simulink model "DPS_LC"  (R2025b)
settings: Solver=FixedStepAuto  StartTime=0.0  StopTime=1  FixedStep=1e-7  RelTol=1e-3
undefined symbols (not defined in the file): Ion, Lithium
libraries: spsVoltageMeasurementLib x5, spsCurrentMeasurementLib x4, spsIGBTDiodeLib x4, spsMosfetLib x4, spsSeriesRLCBranchLib x4, spsDCVoltageSourceLib x2, spsMeanLib x2, spsBatteryLib x1, spsLinearTransformerLib x1, sps_lib x1
settings Model: Creator=photortist  LastModifiedBy=Admin

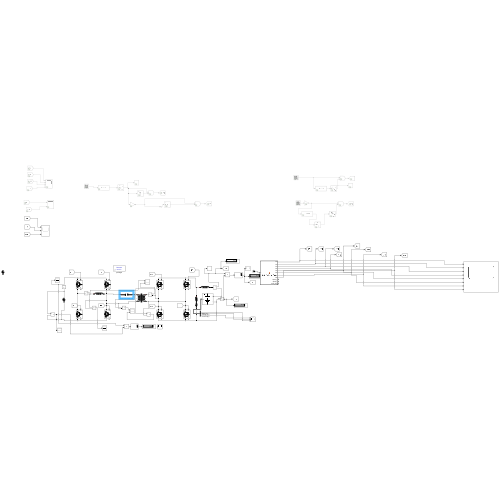
[thumbnail: Simulink's stored preview of the top-level diagram]
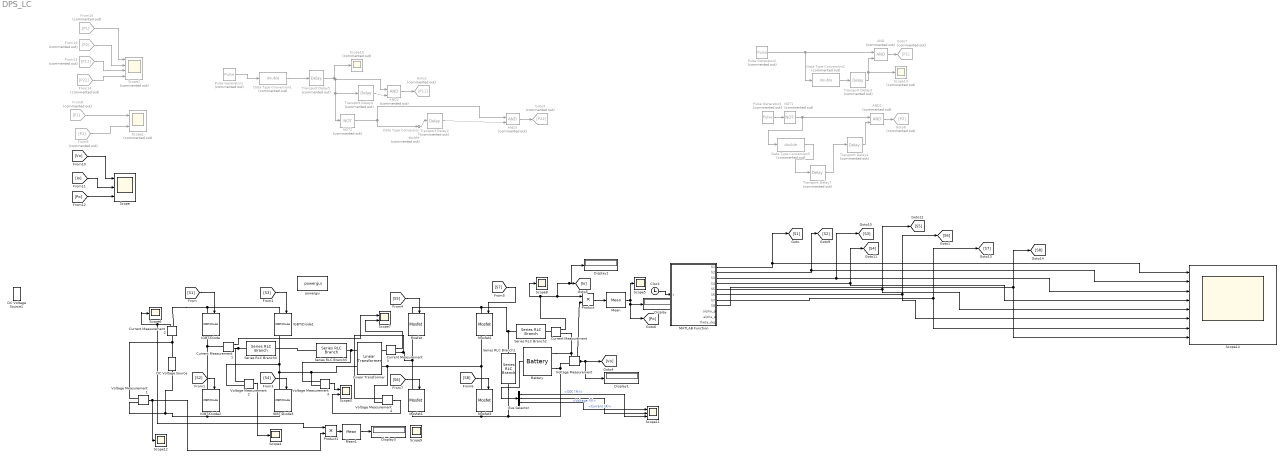
== system DPS_LC ==
  AND{,1..3} (4 alike) : Logic  Commented=on  IconShape=distinctive  AllPortsSameDT=off  OutDataTypeStr=boolean
  Battery : spsBatteryLib/Battery  BatType=Lithium-Ion  NomV=24  NomQ=100  SOC=10  Batt_Tr=0.1  PresetModel=on  MaxQ=100  MinV=18  FullV=27.9357  Dis_rate=43.4783  R=0.0024  Normal_OP=90.4348  expZone="[25.9293      4.91304]"
  Bus Selector : BusSelector  OutputSignals=SOC (%),Voltage (V),Current (A)
  Clock : Clock
  Current Measurement{,1..3} (4 alike) : spsCurrentMeasurementLib/Current Measurement  PhasorSimulation=off  OutputType=Complex  PSBequivalent=0
  DC Voltage Source : spsDCVoltageSourceLib/DC Voltage Source  Amplitude=504  Measurements=None
  DC Voltage Source1 : spsDCVoltageSourceLib/DC Voltage Source  Amplitude=504  Measurements=None
  Data Type Conversion{1..3,5} (4 alike) : DataTypeConversion  Commented=on  OutDataTypeStr=double  SaturateOnIntegerOverflow=off  RndMeth=Floor
  Display{,1..3} (4 alike) : Display
  From13 : From  Commented=on  GotoTag=P11
  From14 : From  Commented=on  GotoTag=P22
  From15 : From  Commented=on  GotoTag=P1
  From16 : From  Commented=on  GotoTag=P2
  From8 : From  Commented=on  GotoTag=P1
  From9 : From  Commented=on  GotoTag=P2
  Goto2 : Goto  Commented=on  GotoTag=P11
  Goto3 : Goto  Commented=on  GotoTag=P22
  Goto7 : Goto  Commented=on  GotoTag=P1
  Goto8 : Goto  Commented=on  GotoTag=P2
  IGBT/Diode{,1..3} (4 alike) : spsIGBTDiodeLib/IGBT//Diode  Ron=1e-4  Rs=1e5  Cs=inf  Measurements=on
  Linear Transformer : spsLinearTransformerLib/Linear Transformer  UNITS=SI  NominalPower=[ 3000 30000 ]  winding1=[504 0 0]  winding2=[28 0 0]  ThreeWindings=off  winding3=[3.15e+05 0.7938 0.084225]  RmLm="[5000  0.05]"  Measurements=None  DataType=on
  MATLAB Function : MATLAB Function  TreatAsAtomicUnit=on
  Mean : spsMeanLib/Mean  Freq=30e3  Vinit=0  Ts=0
  Mean1 : spsMeanLib/Mean  Freq=30e3  Vinit=0  Ts=0
  Mosfet{,1..3} (4 alike) : spsMosfetLib/Mosfet  Ron=1e-4  Lon=0  Rd=0.01  Vfd=0  IC=0  Rs=1e5  Cs=inf  Measurements=on
  NOT1 : Logic  Commented=on  Operator=NOT  IconShape=distinctive  AllPortsSameDT=off  OutDataTypeStr=boolean
  NOT2 : Logic  Commented=on  Operator=NOT  IconShape=distinctive  AllPortsSameDT=off  OutDataTypeStr=boolean
  Product : Product
  Product1 : Product
  Pulse Generator1 : DiscretePulseGenerator  Commented=on  PulseType=Time based  Period=1/30000  PulseWidth=50  PhaseDelay=16.67e-6
  Pulse Generator2 : DiscretePulseGenerator  Commented=on  PulseType=Time based  Period=1/30000  PulseWidth=50  VectorParams1D=off
  Pulse Generator4 : DiscretePulseGenerator  Commented=on  PulseType=Time based  Period=1/30000  PulseWidth=50  VectorParams1D=off
  Scope : Scope  NumInputPorts=3
      settings: Title=Output Voltage  ActiveDisplayYMinimum=-3.1740035321909232  ActiveDisplayYMaximum=28.566031789718316
  Scope1 : Scope  Commented=on  NumInputPorts=2
      settings: ActiveDisplayYMinimum=-1  ActiveDisplayYMaximum=1
  Scope10 : Scope  Commented=on
      settings: ActiveDisplayYMinimum=-0.12499999999999997  ActiveDisplayYMaximum=1.125  DataLoggingVariableName=ScopeData10
  Scope11 : Scope  NumInputPorts=3
      settings: ActiveDisplayYMinimum=-34.642469319088491  ActiveDisplayYMaximum=273.73320486745138  DataLoggingVariableName=ScopeData11
  Scope{4..6,8..9,12} (6 alike) : Scope
      Scope12 settings: ActiveDisplayYMinimum=404  ActiveDisplayYMaximum=604  DataLoggingVariableName=ScopeData12
      Scope4 settings: ActiveDisplayYMinimum=-630.02715891615526  ActiveDisplayYMaximum=630.02739265310572  DataLoggingVariableName=ScopeData4
      Scope5 settings: ActiveDisplayYMinimum=-393.10954952872225  ActiveDisplayYMaximum=3537.9859457585012  DataLoggingVariableName=ScopeData5
      Scope6 settings: ActiveDisplayYMinimum=-23.635845868791428  ActiveDisplayYMaximum=24.862575673067333  DataLoggingVariableName=ScopeData6
      Scope8 settings: ActiveDisplayYMinimum=-843.85888992789546  ActiveDisplayYMaximum=389.64380681826373  DataLoggingVariableName=ScopeData8
      Scope9 settings: ActiveDisplayYMinimum=-44.04044538673373  ActiveDisplayYMaximum=46.396500117844894  DataLoggingVariableName=ScopeData9
  Scope13 : Scope  Commented=on
      settings: ActiveDisplayYMinimum=-0.12499999999999997  ActiveDisplayYMaximum=1.125  DataLoggingVariableName=ScopeData13
  Scope14 : Scope  NumInputPorts=8
      settings: ActiveDisplayYMinimum=-0.12499999999999997  ActiveDisplayYMaximum=1.125  DataLoggingVariableName=ScopeData14
  Scope2 : Scope  Commented=on  NumInputPorts=4
      settings: ActiveDisplayYMinimum=-0.12499999999999997  ActiveDisplayYMaximum=1.125  DataLoggingVariableName=ScopeData2
  Scope3 : Scope  NumInputPorts=2
      settings: ActiveDisplayYMinimum=-1348.3166244930978  ActiveDisplayYMaximum=1342.78051192566  DataLoggingVariableName=ScopeData3
  Scope7 : Scope  NumInputPorts=2
      settings: ActiveDisplayYMinimum=-55.436527647349514  ActiveDisplayYMaximum=40.992607448281404  DataLoggingVariableName=ScopeData7
  Series RLC Branch1 : spsSeriesRLCBranchLib/Series RLC Branch  LConnTagsString=__new0  RConnTagsString=__new0  BranchType=RC  Resistance=0.2  Inductance=1e-3  SetiL0=off  InitialCurrent=0  Capacitance=0.226e-6  Setx0=off  InitialVoltage=0  Measurements=None
  Series RLC Branch2 : spsSeriesRLCBranchLib/Series RLC Branch  LConnTagsString=__new0  RConnTagsString=__new0  BranchType=L  Resistance=7  Inductance=0.5e-6  SetiL0=off  InitialCurrent=0  Capacitance=1e-6  Setx0=off  InitialVoltage=0  Measurements=None
  Series RLC Branch4 : spsSeriesRLCBranchLib/Series RLC Branch  LConnTagsString=__new0  RConnTagsString=__new0  BranchType=L  Resistance=1  Inductance=40e-6  SetiL0=off  InitialCurrent=0  Capacitance=1e-6  Setx0=off  InitialVoltage=0  Measurements=None
  Series RLC Branch5 : spsSeriesRLCBranchLib/Series RLC Branch  LConnTagsString=__new0  RConnTagsString=__new0  BranchType=C  Resistance=0.01  Inductance=350e-6  SetiL0=off  InitialCurrent=0  Capacitance=80.8e-6  Setx0=off  InitialVoltage=0  Measurements=None
  Transport Delay{2..4,6..7} (5 alike) : TransportDelay  Commented=on  DelayTime=0.2e-6
  Transport Delay5 : TransportDelay  Commented=on  DelayTime=16.67e-6
  Voltage Measurement{,1..4} (5 alike) : spsVoltageMeasurementLib/Voltage Measurement  PhasorSimulation=off  OutputType=Complex  PSBequivalent=0
  powergui : sps_lib/powergui  Priority=1  SimulationMode=Discrete  SampleTime=0.1e-6  frequency=60  Iterations=50  frequencyindice=0  Pbase=100e6  ErrMax=1e-4  UnitsV=kV  UnitsW=MW  buscounter=0  FunctionMessages=off  echomessages=off  EnableUseOfTLC=off  CurrentSourceSwitches=off  DisableSnubberDevices=off  DisableRonSwitches=off  DisableVfSwitches=off  DisplayEquations=off  AutomaticDiscreteSolvers=off  SolverType=Tustin/Backward Euler (TBE)  Interpol=off  ExternalGateDelay=off  methode=off  Ts=100  x0status=blocks  SPID=on  SwTol=0  HookPort=off  NonlinearTolerance=1e-4  nMaxIteration=100  ContinueOnMaxIteration=off  RestoreLinks=warning  ResistiveCurrentMeasurement=off  Frange=[0:2:500]  Ylog=off  Xlog=on  ShowGrid=off  save=off  variable=ZData  structure=0  ZoomFFT=off  StartTime=0.0  cycles=1  DisplayStyle=1  fundamental=60  FreqAxis=off  MaxFrequency=1000  frequencyindicesteady=1  RmsSteady=1  display=off
  wires:
  Current Measurement2/1 -> Product1/1, Scope6/1
  Product/1 -> Mean/1
  [Vo] -> Scope/1
  [S2] -> IGBT/Diode2/1
  [S4] -> IGBT/Diode3/1
  [S6] -> Mosfet1/1
  Mean1/1 -> Display3/1
  Voltage Measurement1/1 -> Scope12/1, Product1/2
  From8/1 -> Scope1/1
  [S3] -> IGBT/Diode1/1
  From9/1 -> Scope1/2
  Current Measurement3/1 -> Scope7/2
  Voltage Measurement2/1 -> Scope4/1
  From14/1 -> Scope2/4
  [S8] -> Mosfet3/1
  Pulse Generator1/1 -> Data Type Conversion1/1
  Current Measurement/1 -> Scope8/1, Product/1, Display2/1, [Io]
  From16/1 -> Scope2/2
  [Io] -> Scope/2
  Mean/1 -> [Po], Display/1, Scope5/1
  [S7] -> Mosfet2/1
  Voltage Measurement3/1 -> Scope3/1
  [S1] -> IGBT/Diode/1
  From15/1 -> Scope2/1
  From13/1 -> Scope2/3
  Product1/1 -> Mean1/1
  Current Measurement1/1 -> Scope7/1
  [S5] -> Mosfet/1
  Voltage Measurement/1 -> Product/2, [Vo], Display1/1
  [Po] -> Scope/3
  Data Type Conversion2/1 -> Transport Delay3/1
  Pulse Generator2/1 -> Data Type Conversion2/1, AND/1
  Transport Delay3/1 -> Scope13/1, AND/2
  Transport Delay4/1 -> AND1/2
  Pulse Generator4/1 -> NOT1/1
  NOT1/1 -> Data Type Conversion3/1, AND1/1
  AND/1 -> Goto7/1
  AND1/1 -> Goto8/1
  NOT2/1 -> AND3/1, Data Type Conversion5/1
  Data Type Conversion1/1 -> Transport Delay5/1
  AND2/1 -> Goto2/1
  Transport Delay6/1 -> AND2/2
  Data Type Conversion5/1 -> Transport Delay2/1
  Transport Delay2/1 -> AND3/2
  AND3/1 -> Goto3/1
  Transport Delay5/1 -> AND2/1, NOT2/1, Transport Delay6/1, Scope10/1
  Data Type Conversion3/1 -> Transport Delay7/1
  Transport Delay7/1 -> Transport Delay4/1
  Voltage Measurement4/1 -> Scope3/2
  Battery/1 -> Bus Selector/1
  Bus Selector/1 -> Scope11/3  "<SOC (%)>"
  Bus Selector/2 -> Scope11/2  "<Voltage (V)>"
  Bus Selector/3 -> Scope11/1  "<Current (A)>"
  MATLAB Function/7(S7) -> [S7], Scope14/7
  MATLAB Function/6(S6) -> [S6], Scope14/6
  MATLAB Function/8(S8) -> Scope14/8, [S8]
  MATLAB Function/3(S3) -> [S3], Scope14/3
  MATLAB Function/5(S5) -> Scope14/5, [S5]
  MATLAB Function/1(S1) -> [S1], Scope14/1
  MATLAB Function/2(S2) -> [S2], Scope14/2
  MATLAB Function/4(S4) -> Scope14/4, [S4]
  Clock/1 -> MATLAB Function/1(t)
  connections:
  Current Measurement2/LConn1 -- DC Voltage Source/RConn1 -- Voltage Measurement1/LConn1
  Current Measurement3/RConn1 -- Mosfet1/LConn1 -- Mosfet/RConn1 -- Voltage Measurement4/LConn1
  Current Measurement1/RConn1 -- Voltage Measurement2/LConn1 -- Series RLC Branch4/LConn1
  Current Measurement/RConn1 -- Battery/LConn1 -- Voltage Measurement/LConn1
  Linear Transformer/RConn2 -- Mosfet3/LConn1 -- Mosfet2/RConn1 -- Voltage Measurement4/LConn2
  Mosfet2/LConn1 -- Series RLC Branch1/LConn1 -- Series RLC Branch2/LConn1 -- Mosfet/LConn1
  IGBT/Diode3/RConn1 -- Voltage Measurement1/LConn2 -- DC Voltage Source/LConn1 -- IGBT/Diode2/RConn1
  Linear Transformer/LConn2 -- IGBT/Diode3/LConn1 -- IGBT/Diode1/RConn1 -- Voltage Measurement2/LConn2 -- Voltage Measurement3/LConn2
  Series RLC Branch5/LConn1 -- Series RLC Branch4/RConn1
  IGBT/Diode1/LConn1 -- Current Measurement2/RConn1 -- IGBT/Diode/LConn1
  IGBT/Diode2/LConn1 -- IGBT/Diode/RConn1 -- Current Measurement1/LConn1
  Linear Transformer/LConn1 -- Voltage Measurement3/LConn1 -- Series RLC Branch5/RConn1
  Linear Transformer/RConn1 -- Current Measurement3/LConn1
  Current Measurement/LConn1 -- Series RLC Branch2/RConn1
  Mosfet1/RConn1 -- Voltage Measurement/LConn2 -- Battery/LConn2 -- Series RLC Branch1/RConn1 -- Mosfet3/RConn1

== matlab function DPS_LC/MATLAB Function ==
  settings: updateMethod=DISCRETE
  data: S1 output; S2 output; S3 output; S4 output; S5 output; S6 output; S7 output; S8 output; t input; alpha_p output; alpha_s output; theta_deg output
function [S1, S2, S3, S4, S5, S6, S7, S8, alpha_p, alpha_s, theta_deg] = DAB_MaxPower_Test(t)
%#codegen
% =========================================================================
% FIXED MAXIMUM POWER TEST: alpha_p = 0 deg, alpha_s = 0 deg, theta = 90 deg
% Switching Frequency: fs = 30 kHz (Ts = 33.3333 us)
% =========================================================================

    % 1. FIXED ANGLES & DIRECTION
    alpha_p   = 5.0;        % Primary inner shift = 0 deg
    alpha_s   = 5.0;        % Secondary inner shift = 0 deg
    theta_deg =5;       % Outer phase shift = 90 deg (Max Power Point)
    DIRECTION = 1.0;        % +1.0 = HV -> LV, -1.0 = LV -> HV

    % 2. TIMING & DEAD-TIME PARAMETERS
    fs      = 30000.0;      % 30 kHz
    Ts      = 1.0 / fs;     % 33.3333 us
    half_Ts = Ts / 2.0;     % 180 deg = 16.6667 us

    dt_hv   = 0.4e-6;       % HV Dead-time = 0.4 us (Ideal test के लिए 0.0 कर सकते हैं)
    dt_lv   = 0.2e-6;       % LV Dead-time = 0.2 us

    % 3. CONVERT ANGLES TO TIME DELAYS
    theta_applied = DIRECTION * theta_deg;
    t_inner_hv    = ((2.0 * alpha_p) / 360.0) * Ts;   % 0 us
    t_inner_lv    = ((2.0 * alpha_s) / 360.0) * Ts;   % 0 us
    t_outer       = (theta_applied / 360.0) * Ts;     % 8.3333 us (Quarter period)

    % 4. CARRIER TIME REFERENCES
    t_hv_L = mod(t, Ts);                                    % HV Left Leg  (S1, S2)
    t_hv_R = mod(t - half_Ts - t_inner_hv, Ts);             % HV Right Leg (S3, S4)

    t_lv_L = mod(t - t_outer, Ts);                          % LV Left Leg  (S5, S6)
    t_lv_R = mod(t - t_outer - half_Ts - t_inner_lv, Ts);   % LV Right Leg (S7, S8)

    % 5. GATE PULSES (HV BRIDGE: S1..S4)
    if (t_hv_L >= dt_hv) && (t_hv_L < half_Ts), S1 = 1; else, S1 = 0; end
    if (t_hv_L >= half_Ts + dt_hv) && (t_hv_L < Ts), S2 = 1; else, S2 = 0; end

    if (t_hv_R >= dt_hv) && (t_hv_R < half_Ts), S3 = 1; else, S3 = 0; end
    if (t_hv_R >= half_Ts + dt_hv) && (t_hv_R < Ts), S4 = 1; else, S4 = 0; end

    % 6. GATE PULSES (LV BRIDGE: S5..S8)
    if (t_lv_L >= dt_lv) && (t_lv_L < half_Ts), S5 = 1; else, S5 = 0; end
    if (t_lv_L >= half_Ts + dt_lv) && (t_lv_L < Ts), S6 = 1; else, S6 = 0; end

    if (t_lv_R >= dt_lv) && (t_lv_R < half_Ts), S7 = 1; else, S7 = 0; end
    if (t_lv_R >= half_Ts + dt_lv) && (t_lv_R < Ts), S8 = 1; else, S8 = 0; end

end
